simulink model "AFC_FFNN_trainlm_45_45_45_ctr_Nor_July_15"  (R2021a)
settings: Solver=VariableStepAuto  StartTime=0.0  StopTime=10.0  RelTol=1e-3
libraries: neural x140
(part 1 of 6)
settings Model: Creator=deyun  LastModifiedBy=deyun

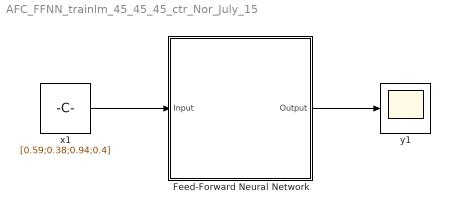
== system AFC_FFNN_trainlm_45_45_45_ctr_Nor_July_15 ==
  Feed-Forward Neural Network : Subsystem
      mask help: Feed-Forward Neural Network
      mask Display: e = 0.06;c1 = [120 150 230]/255;c2 = ([120 150 230]+0)/383;c3 = ([120 150 230]+128)/383;patch([0 1 1 0],[0 0 1 1],c1);patch([0 1 1 1-e 1-e 0+e],[0 0 1 1-e 0+e 0+e],c2);patch([0 0 1 1-e 0+e 0+e],[0 1 1 1-e 1-e 0+e],c3);plot([0 1 1 0 0],[0 0 1 1 0]);fprintf('NNET');port_label('input',1,' Input');port_label('output',1,'Output ');
  x1 : Constant  Value=[0.59;0.38;0.94;0.4]  SampleTime=1
      mask Display: e = 0.06;c1 = [120 230 180]/255;c2 = ([120 230 180]+0)/(256+128);c3 = ([120 230 180]+128)/(256+128);patch([0 1 1 0],[0 0 1 1],c1);patch([0 1 1 1-e 1-e 0+e],[0 0 1 1-e 0+e 0+e],c2);patch([0 0 1 1-e 0+e 0+e],[0 1 1 1-e 1-e 0+e],c3);plot([0 1 1 0 0],[0 0 1 1 0]);disp('Constant');
  y1 : Scope
      mask Display: e = 0.06;c1 = [120 230 180]/255;c2 = ([120 230 180]+0)/(256+128);c3 = ([120 230 180]+128)/(256+128);patch([0 1 1 0],[0 0 1 1],c1);patch([0 1 1 1-e 1-e 0+e],[0 0 1 1-e 0+e 0+e],c2);patch([0 0 1 1-e 0+e 0+e],[0 1 1 1-e 1-e 0+e],c3);plot([0 1 1 0 0],[0 0 1 1 0]);plot([0.15 0.85 0.85 0.15 0.15],[0.5 0.5 0.85 0.85 0.5]);
  wires:
  x1/1 -> Feed-Forward Neural Network/1(Input)
  Feed-Forward Neural Network/1(Output) -> y1/1

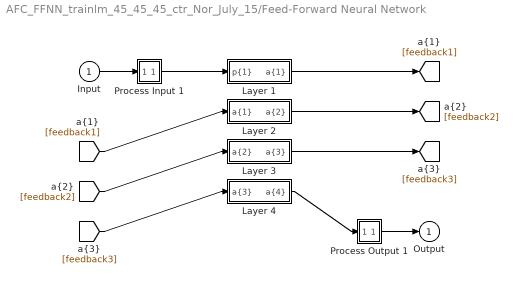
== system AFC_FFNN_trainlm_45_45_45_ctr_Nor_July_15/Feed-Forward Neural Network ==
  Input : Inport  PortDimensions=4
      mask Display: e = 0.06;c1 = [120 230 180]/255;c2 = ([120 230 180]+0)/(256+128);c3 = ([120 230 180]+128)/(256+128);patch([0 1 1 0],[0 0 1 1],c1);patch([0 1 1 1-e 1-e 0+e],[0 0 1 1-e 0+e 0+e],c2);patch([0 0 1 1-e 0+e 0+e],[0 1 1 1-e 1-e 0+e],c3);plot([0 1 1 0 0],[0 0 1 1 0]);
  Layer 1 : Subsystem
      mask Display: e = 0.06;c1 = [120 150 230]/255;c2 = ([120 150 230]+0)/383;c3 = ([120 150 230]+128)/383;patch([0 1 1 0],[0 0 1 1],c1);patch([0 1 1 1-e 1-e 0+e],[0 0 1 1-e 0+e 0+e],c2);patch([0 0 1 1-e 0+e 0+e],[0 1 1 1-e 1-e 0+e],c3);plot([0 1 1 0 0],[0 0 1 1 0]);
  Layer 2 : Subsystem
      mask Display: e = 0.06;c1 = [120 150 230]/255;c2 = ([120 150 230]+0)/383;c3 = ([120 150 230]+128)/383;patch([0 1 1 0],[0 0 1 1],c1);patch([0 1 1 1-e 1-e 0+e],[0 0 1 1-e 0+e 0+e],c2);patch([0 0 1 1-e 0+e 0+e],[0 1 1 1-e 1-e 0+e],c3);plot([0 1 1 0 0],[0 0 1 1 0]);
  Layer 3 : Subsystem
      mask Display: e = 0.06;c1 = [120 150 230]/255;c2 = ([120 150 230]+0)/383;c3 = ([120 150 230]+128)/383;patch([0 1 1 0],[0 0 1 1],c1);patch([0 1 1 1-e 1-e 0+e],[0 0 1 1-e 0+e 0+e],c2);patch([0 0 1 1-e 0+e 0+e],[0 1 1 1-e 1-e 0+e],c3);plot([0 1 1 0 0],[0 0 1 1 0]);
  Layer 4 : Subsystem
      mask Display: e = 0.06;c1 = [120 150 230]/255;c2 = ([120 150 230]+0)/383;c3 = ([120 150 230]+128)/383;patch([0 1 1 0],[0 0 1 1],c1);patch([0 1 1 1-e 1-e 0+e],[0 0 1 1-e 0+e 0+e],c2);patch([0 0 1 1-e 0+e 0+e],[0 1 1 1-e 1-e 0+e],c3);plot([0 1 1 0 0],[0 0 1 1 0]);
  Process Input 1 : Subsystem
      mask Display: e = 0.06;c1 = [120 150 230]/255;c2 = ([120 150 230]+0)/383;c3 = ([120 150 230]+128)/383;patch([0 1 1 0],[0 0 1 1],c1);patch([0 1 1 1-e 1-e 0+e],[0 0 1 1-e 0+e 0+e],c2);patch([0 0 1 1-e 0+e 0+e],[0 1 1 1-e 1-e 0+e],c3);plot([0 1 1 0 0],[0 0 1 1 0]);
  Process Output 1 : Subsystem
      mask Display: e = 0.06;c1 = [120 150 230]/255;c2 = ([120 150 230]+0)/383;c3 = ([120 150 230]+128)/383;patch([0 1 1 0],[0 0 1 1],c1);patch([0 1 1 1-e 1-e 0+e],[0 0 1 1-e 0+e 0+e],c2);patch([0 0 1 1-e 0+e 0+e],[0 1 1 1-e 1-e 0+e],c3);plot([0 1 1 0 0],[0 0 1 1 0]);
  Output : Outport  InitialOutput=0
      mask Display: e = 0.06;c1 = [120 230 180]/255;c2 = ([120 230 180]+0)/(256+128);c3 = ([120 230 180]+128)/(256+128);patch([0 1 1 0],[0 0 1 1],c1);patch([0 1 1 1-e 1-e 0+e],[0 0 1 1-e 0+e 0+e],c2);patch([0 0 1 1-e 0+e 0+e],[0 1 1 1-e 1-e 0+e],c3);plot([0 1 1 0 0],[0 0 1 1 0]);
  wires:
  Input/1 -> Process Input 1/1(x)
  Process Output 1/1(y) -> Output/1
  Process Input 1/1(p) -> Layer 1/1("p{1}")
  Layer 1/1("a{1}") -> [feedback1]
  [feedback1] -> Layer 2/1("a{1} ")
  Layer 2/1("a{2}") -> [feedback2]
  [feedback2] -> Layer 3/1("a{2} ")
  Layer 3/1("a{3}") -> [feedback3]
  [feedback3] -> Layer 4/1("a{3} ")
  Layer 4/1("a{4}") -> Process Output 1/1(a)

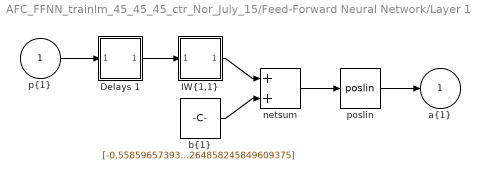
== system AFC_FFNN_trainlm_45_45_45_ctr_Nor_July_15/Feed-Forward Neural Network/Layer 1 ==
  "p{1}" : Inport  PortDimensions=4
      mask Display: e = 0.06;c1 = [120 230 180]/255;c2 = ([120 230 180]+0)/(256+128);c3 = ([120 230 180]+128)/(256+128);patch([0 1 1 0],[0 0 1 1],c1);patch([0 1 1 1-e 1-e 0+e],[0 0 1 1-e 0+e 0+e],c2);patch([0 0 1 1-e 0+e 0+e],[0 1 1 1-e 1-e 0+e],c3);plot([0 1 1 0 0],[0 0 1 1 0]);
  Delays 1 : Subsystem
      mask Display: e = 0.06;c1 = [120 150 230]/255;c2 = ([120 150 230]+0)/383;c3 = ([120 150 230]+128)/383;patch([0 1 1 0],[0 0 1 1],c1);patch([0 1 1 1-e 1-e 0+e],[0 0 1 1-e 0+e 0+e],c2);patch([0 0 1 1-e 0+e 0+e],[0 1 1 1-e 1-e 0+e],c3);plot([0 1 1 0 0],[0 0 1 1 0]);disp('0');
  "IW{1,1}" : Subsystem
      mask Display: e = 0.06;c1 = [120 150 230]/255;c2 = ([120 150 230]+0)/383;c3 = ([120 150 230]+128)/383;patch([0 1 1 0],[0 0 1 1],c1);patch([0 1 1 1-e 1-e 0+e],[0 0 1 1-e 0+e 0+e],c2);patch([0 0 1 1-e 0+e 0+e],[0 1 1 1-e 1-e 0+e],c3);plot([0 1 1 0 0],[0 0 1 1 0]);disp('W');
  "b{1}" : Constant  Value=[-0.5585965739320057910077821361483074724674224853515625;-0.77112950387139012065063070622272789478302001953125;0.22894666757716020111246280066552571952342987060546875;-0.305047379583083699827739110332913696765899658203125;-0.69451441467543661989481051932671107351779937744140625;0.39214635280524723359718564097420312464237213134765625;-0.1555721937487436756786252090023481287062168121337890625;0.274827394729951490770503141902736388146877288818359375;0.277365245819692296525005303919897414743900299072265625;-0.1524186026109950187201746985010686330497264862060546875;-0.0018307247949869154268753845826722681522369384765625;0.58822997451524916545650967236724682152271270751953125;0.55084837701463318371253308214363642036914825439453125;0.314130170445041712046219117837608791887760162353515625;-0.07693509824360840465562461076842737384140491485595703125;-0.851136421274869547914931899867951869964599609375;0.362298342175110754670441792768542654812335968017578125;0.21255578744349323816464902847656048834323883056640625;-0.3824877228684744334685774447279982268810272216796875;-0.6749591132024963524571603556978516280651092529296875;-0.63890547966722144312967657242552377283573150634765625;-0.149732930796697971675968119598110206425189971923828125;-0.933207190422134402751908055506646633148193359375;0.10402318613955320592001640989110455848276615142822265625;0.829936502547987675626472992007620632648468017578125;-0.737888972575629242811601216089911758899688720703125;0.21732415928306558772220569153432734310626983642578125;-0.1580532967861125737130123525275848805904388427734375;-1.288298758066100280217369800084270536899566650390625;-0.9481540190806569956549765265663154423236846923828125;0.942806016112406108931054404820315539836883544921875;-0.439159443551665196192601570146507583558559417724609375;0.276425093592411907916783775363001041114330291748046875;0.485464567417084047473707641984219662845134735107421875;0.295746825087029263645632681800634600222110748291015625;-0.8382271786519968070905406420934014022350311279296875;-0.1591390063283328881738043492077849805355072021484375;-0.7823304156725818803153060798649676144123077392578125;0.2224216466664273028630560702367802150547504425048828125;0.75721224172485557257772370576276443898677825927734375;-0.26127862544034818892413341018254868686199188232421875;0.1681522472301393289484394699684344232082366943359375;0.00998894613673773079653983586467802524566650390625;-0.6614665456480552929718896848498843610286712646484375;-0.838290046288482582070855642086826264858245849609375]
      mask Display: e = 0.06;c1 = [120 150 230]/255;c2 = ([120 150 230]+0)/383;c3 = ([120 150 230]+128)/383;patch([0 1 1 0],[0 0 1 1],c1);patch([0 1 1 1-e 1-e 0+e],[0 0 1 1-e 0+e 0+e],c2);patch([0 0 1 1-e 0+e 0+e],[0 1 1 1-e 1-e 0+e],c3);plot([0 1 1 0 0],[0 0 1 1 0]);disp('b');
  netsum : Sum  Inputs=2  InputSameDT=on  SaturateOnIntegerOverflow=on  OutDataTypeStr=Inherit: Same as first input
      mask Display: e = 0.06;c1 = [120 150 230]/255;c2 = ([120 150 230]+0)/383;c3 = ([120 150 230]+128)/383;patch([0 1 1 0],[0 0 1 1],c1);patch([0 1 1 1-e 1-e 0+e],[0 0 1 1-e 0+e 0+e],c2);patch([0 0 1 1-e 0+e 0+e],[0 1 1 1-e 1-e 0+e],c3);plot([0 1 1 0 0],[0 0 1 1 0]);disp('+');
  poslin : neural/Transfer Functions/poslin
      settings: SourceProductBaseCode=NN
  "a{1}" : Outport  InitialOutput=[0;0;0;0;0;0;0;0;0;0;0;0;0;0;0;0;0;0;0;0;0;0;0;0;0;0;0;0;0;0;0;0;0;0;0;0;0;0;0;0;0;0;0;0;0]
      mask Display: e = 0.06;c1 = [120 230 180]/255;c2 = ([120 230 180]+0)/(256+128);c3 = ([120 230 180]+128)/(256+128);patch([0 1 1 0],[0 0 1 1],c1);patch([0 1 1 1-e 1-e 0+e],[0 0 1 1-e 0+e 0+e],c2);patch([0 0 1 1-e 0+e 0+e],[0 1 1 1-e 1-e 0+e],c3);plot([0 1 1 0 0],[0 0 1 1 0]);
  wires:
  "p{1}"/1 -> Delays 1/1("p{1}")
  Delays 1/1("pd{1,1}") -> "IW{1,1}"/1("pd{1,1}")
  "IW{1,1}"/1("iz{1,1}") -> netsum/1
  "b{1}"/1 -> netsum/2
  netsum/1 -> poslin/1
  poslin/1 -> "a{1}"/1

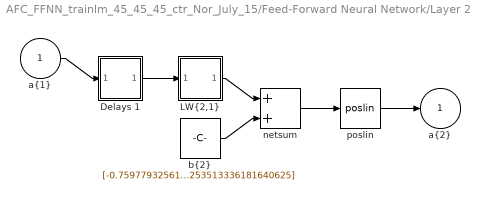
== system AFC_FFNN_trainlm_45_45_45_ctr_Nor_July_15/Feed-Forward Neural Network/Layer 2 ==
  "a{1} " : Inport  PortDimensions=45
      mask Display: e = 0.06;c1 = [120 230 180]/255;c2 = ([120 230 180]+0)/(256+128);c3 = ([120 230 180]+128)/(256+128);patch([0 1 1 0],[0 0 1 1],c1);patch([0 1 1 1-e 1-e 0+e],[0 0 1 1-e 0+e 0+e],c2);patch([0 0 1 1-e 0+e 0+e],[0 1 1 1-e 1-e 0+e],c3);plot([0 1 1 0 0],[0 0 1 1 0]);
  Delays 1 : Subsystem
      mask Display: e = 0.06;c1 = [120 150 230]/255;c2 = ([120 150 230]+0)/383;c3 = ([120 150 230]+128)/383;patch([0 1 1 0],[0 0 1 1],c1);patch([0 1 1 1-e 1-e 0+e],[0 0 1 1-e 0+e 0+e],c2);patch([0 0 1 1-e 0+e 0+e],[0 1 1 1-e 1-e 0+e],c3);plot([0 1 1 0 0],[0 0 1 1 0]);disp('0');
  "LW{2,1}" : Subsystem
      mask Display: e = 0.06;c1 = [120 150 230]/255;c2 = ([120 150 230]+0)/383;c3 = ([120 150 230]+128)/383;patch([0 1 1 0],[0 0 1 1],c1);patch([0 1 1 1-e 1-e 0+e],[0 0 1 1-e 0+e 0+e],c2);patch([0 0 1 1-e 0+e 0+e],[0 1 1 1-e 1-e 0+e],c3);plot([0 1 1 0 0],[0 0 1 1 0]);disp('W');
  "b{2}" : Constant  Value=[-0.759779325613544553874589837505482137203216552734375;0.6965202526642186864336281360010616481304168701171875;-0.861179161880855748023577689309604465961456298828125;0.279069361418990080636604034225456416606903076171875;0.7788995695670519747721982639632187783718109130859375;0.72059847295826762181292224340722896158695220947265625;0.56823299771985691375419946780311875045299530029296875;-0.814016852489903186551600811071693897247314453125;-0.25020043213131148984729179574060253798961639404296875;0.3676809986895264170669861414353363215923309326171875;-0.5664709440966280151741329973447136580944061279296875;0.02629409189089770837455262153525836765766143798828125;-0.54936854809591240123012312324135564267635345458984375;-0.133862432529689490134927609688020311295986175537109375;-0.81332808228198449906898304107016883790493011474609375;-0.75199519420301730310285392988589592278003692626953125;-1.0530530335707963818236976294429041445255279541015625;-0.3949760005903317772180116662639193236827850341796875;0.08349711700445057449559982387654599733650684356689453125;-0.5150947870913196169340153574012219905853271484375;0.80569296901346032502289062904310412704944610595703125;-0.335455649950676171311414464071276597678661346435546875;0.2177777173381762187975851929877535440027713775634765625;-0.24227916035240870673561630610493011772632598876953125;-0.7581191909009616924919328084797598421573638916015625;-0.316127694986459373271969752750010229647159576416015625;-0.7572608648365470873642379956436343491077423095703125;-0.1771784549431406896591312261080020107328891754150390625;0.6700945036965897383396395525778643786907196044921875;-0.37793060271353240420211250238935463130474090576171875;0.49989124604212953340010017200256697833538055419921875;-0.8804292366841608430405585750122554600238800048828125;-0.68894262263308225779923077425337396562099456787109375;-0.7835754927496629829164476177538745105266571044921875;-0.331990649298899709318533268742612563073635101318359375;-0.365329678636181875983623967840685509145259857177734375;-0.1674592513076313959885510485037229955196380615234375;-0.65902586680079677794452663874835707247257232666015625;-0.045949912742535292675682967455941252410411834716796875;-0.56660135380107534697202709139673970639705657958984375;0.85478289689744979540364511194638907909393310546875;0.8907503577019373341983055070159025490283966064453125;-0.7442862631882911639280564486398361623287200927734375;0.8790617462862424513758696775767020881175994873046875;-0.487941954201235095212041414924897253513336181640625]
      mask Display: e = 0.06;c1 = [120 150 230]/255;c2 = ([120 150 230]+0)/383;c3 = ([120 150 230]+128)/383;patch([0 1 1 0],[0 0 1 1],c1);patch([0 1 1 1-e 1-e 0+e],[0 0 1 1-e 0+e 0+e],c2);patch([0 0 1 1-e 0+e 0+e],[0 1 1 1-e 1-e 0+e],c3);plot([0 1 1 0 0],[0 0 1 1 0]);disp('b');
  netsum : Sum  Inputs=2  InputSameDT=on  SaturateOnIntegerOverflow=on  OutDataTypeStr=Inherit: Same as first input
      mask Display: e = 0.06;c1 = [120 150 230]/255;c2 = ([120 150 230]+0)/383;c3 = ([120 150 230]+128)/383;patch([0 1 1 0],[0 0 1 1],c1);patch([0 1 1 1-e 1-e 0+e],[0 0 1 1-e 0+e 0+e],c2);patch([0 0 1 1-e 0+e 0+e],[0 1 1 1-e 1-e 0+e],c3);plot([0 1 1 0 0],[0 0 1 1 0]);disp('+');
  poslin : neural/Transfer Functions/poslin
      settings: SourceProductBaseCode=NN
  "a{2}" : Outport  InitialOutput=[0;0;0;0;0;0;0;0;0;0;0;0;0;0;0;0;0;0;0;0;0;0;0;0;0;0;0;0;0;0;0;0;0;0;0;0;0;0;0;0;0;0;0;0;0]
      mask Display: e = 0.06;c1 = [120 230 180]/255;c2 = ([120 230 180]+0)/(256+128);c3 = ([120 230 180]+128)/(256+128);patch([0 1 1 0],[0 0 1 1],c1);patch([0 1 1 1-e 1-e 0+e],[0 0 1 1-e 0+e 0+e],c2);patch([0 0 1 1-e 0+e 0+e],[0 1 1 1-e 1-e 0+e],c3);plot([0 1 1 0 0],[0 0 1 1 0]);
  wires:
  "a{1} "/1 -> Delays 1/1("p{2}")
  Delays 1/1("pd{2,1}") -> "LW{2,1}"/1("ad{2,1}")
  "LW{2,1}"/1("lz{2,1}") -> netsum/1
  "b{2}"/1 -> netsum/2
  netsum/1 -> poslin/1
  poslin/1 -> "a{2}"/1

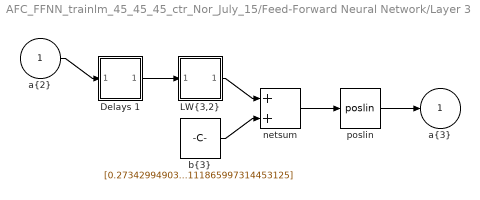
== system AFC_FFNN_trainlm_45_45_45_ctr_Nor_July_15/Feed-Forward Neural Network/Layer 3 ==
  "a{2} " : Inport  PortDimensions=45
      mask Display: e = 0.06;c1 = [120 230 180]/255;c2 = ([120 230 180]+0)/(256+128);c3 = ([120 230 180]+128)/(256+128);patch([0 1 1 0],[0 0 1 1],c1);patch([0 1 1 1-e 1-e 0+e],[0 0 1 1-e 0+e 0+e],c2);patch([0 0 1 1-e 0+e 0+e],[0 1 1 1-e 1-e 0+e],c3);plot([0 1 1 0 0],[0 0 1 1 0]);
  Delays 1 : Subsystem
      mask Display: e = 0.06;c1 = [120 150 230]/255;c2 = ([120 150 230]+0)/383;c3 = ([120 150 230]+128)/383;patch([0 1 1 0],[0 0 1 1],c1);patch([0 1 1 1-e 1-e 0+e],[0 0 1 1-e 0+e 0+e],c2);patch([0 0 1 1-e 0+e 0+e],[0 1 1 1-e 1-e 0+e],c3);plot([0 1 1 0 0],[0 0 1 1 0]);disp('0');
  "LW{3,2}" : Subsystem
      mask Display: e = 0.06;c1 = [120 150 230]/255;c2 = ([120 150 230]+0)/383;c3 = ([120 150 230]+128)/383;patch([0 1 1 0],[0 0 1 1],c1);patch([0 1 1 1-e 1-e 0+e],[0 0 1 1-e 0+e 0+e],c2);patch([0 0 1 1-e 0+e 0+e],[0 1 1 1-e 1-e 0+e],c3);plot([0 1 1 0 0],[0 0 1 1 0]);disp('W');
  "b{3}" : Constant  Value=[0.2734299490328331305732945111230947077274322509765625;0.253212645186324747381689803660265170037746429443359375;0.93467329178748126405906759828212670981884002685546875;0.85424049495533072029473942166077904403209686279296875;0.370732482252811246237200748510076664388179779052734375;0.58575586111893096497027499935938976705074310302734375;-0.57222729704926555971411517020897008478641510009765625;0.402075725104235726092838376644067466259002685546875;0.77510392535672212321884444463648833334445953369140625;0.89750677439359172193888980473275296390056610107421875;-0.53893848136911326474063343994203023612499237060546875;-0.447084590177655893938890585559420287609100341796875;-0.16971363346798085114386367422412149608135223388671875;-0.1253386080403514346581772542776889167726039886474609375;0.7324385856904609415352069845539517700672149658203125;-0.1718566614749994225785911794446292333304882049560546875;-0.649121257858855216227311757393181324005126953125;0.0020706443178506819292883367467084099189378321170806884765625;0.14280132148982105366741279794950969517230987548828125;-0.400326950100625911233009901479817926883697509765625;-0.09611968684726655831607189384158118627965450286865234375;-0.86780297012492602082289749887422658503055572509765625;-0.22662709591045449020185742483590729534626007080078125;-0.049925910120531102887042607108014635741710662841796875;0.957436543865733735714229624136351048946380615234375;0.557449966972769939133058869629167020320892333984375;-0.28645987977858933248853645636700093746185302734375;0.1261192693375135787103857865076861344277858734130859375;-0.5205296579813223356580920153646729886531829833984375;0.30033442526422593488177881226874887943267822265625;-0.17988670535213813206354416251997463405132293701171875;0.88536176329107918459015991174965165555477142333984375;0.52550652298814781726576939036021940410137176513671875;0.55963934687581906590736480211489833891391754150390625;0.1453135731776866723663488301099278032779693603515625;0.5122265681069091414201466250233352184295654296875;-0.3700450504693375552989209609222598373889923095703125;0.0395997938226071710676734483058680780231952667236328125;0.741921262418416826989187029539607465267181396484375;-0.1478710785470286614984303241726593114435672760009765625;0.3344458719405338786856418664683587849140167236328125;-0.562784675088596753056435773032717406749725341796875;0.6146888018342695492179927896359004080295562744140625;0.41510836491622049582161935177282430231571197509765625;0.885843136212703274878776937839575111865997314453125]
      mask Display: e = 0.06;c1 = [120 150 230]/255;c2 = ([120 150 230]+0)/383;c3 = ([120 150 230]+128)/383;patch([0 1 1 0],[0 0 1 1],c1);patch([0 1 1 1-e 1-e 0+e],[0 0 1 1-e 0+e 0+e],c2);patch([0 0 1 1-e 0+e 0+e],[0 1 1 1-e 1-e 0+e],c3);plot([0 1 1 0 0],[0 0 1 1 0]);disp('b');
  netsum : Sum  Inputs=2  InputSameDT=on  SaturateOnIntegerOverflow=on  OutDataTypeStr=Inherit: Same as first input
      mask Display: e = 0.06;c1 = [120 150 230]/255;c2 = ([120 150 230]+0)/383;c3 = ([120 150 230]+128)/383;patch([0 1 1 0],[0 0 1 1],c1);patch([0 1 1 1-e 1-e 0+e],[0 0 1 1-e 0+e 0+e],c2);patch([0 0 1 1-e 0+e 0+e],[0 1 1 1-e 1-e 0+e],c3);plot([0 1 1 0 0],[0 0 1 1 0]);disp('+');
  poslin : neural/Transfer Functions/poslin
      settings: SourceProductBaseCode=NN
  "a{3}" : Outport  InitialOutput=[0;0;0;0;0;0;0;0;0;0;0;0;0;0;0;0;0;0;0;0;0;0;0;0;0;0;0;0;0;0;0;0;0;0;0;0;0;0;0;0;0;0;0;0;0]
      mask Display: e = 0.06;c1 = [120 230 180]/255;c2 = ([120 230 180]+0)/(256+128);c3 = ([120 230 180]+128)/(256+128);patch([0 1 1 0],[0 0 1 1],c1);patch([0 1 1 1-e 1-e 0+e],[0 0 1 1-e 0+e 0+e],c2);patch([0 0 1 1-e 0+e 0+e],[0 1 1 1-e 1-e 0+e],c3);plot([0 1 1 0 0],[0 0 1 1 0]);
  wires:
  "a{2} "/1 -> Delays 1/1("p{3}")
  Delays 1/1("pd{3,2}") -> "LW{3,2}"/1("ad{3,2}")
  "LW{3,2}"/1("lz{3,2}") -> netsum/1
  "b{3}"/1 -> netsum/2
  netsum/1 -> poslin/1
  poslin/1 -> "a{3}"/1

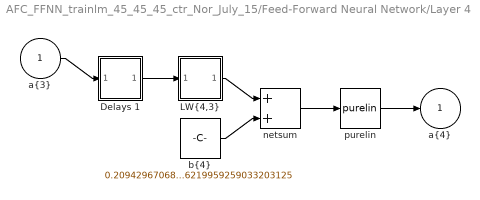
== system AFC_FFNN_trainlm_45_45_45_ctr_Nor_July_15/Feed-Forward Neural Network/Layer 4 ==
  "a{3} " : Inport  PortDimensions=45
      mask Display: e = 0.06;c1 = [120 230 180]/255;c2 = ([120 230 180]+0)/(256+128);c3 = ([120 230 180]+128)/(256+128);patch([0 1 1 0],[0 0 1 1],c1);patch([0 1 1 1-e 1-e 0+e],[0 0 1 1-e 0+e 0+e],c2);patch([0 0 1 1-e 0+e 0+e],[0 1 1 1-e 1-e 0+e],c3);plot([0 1 1 0 0],[0 0 1 1 0]);
  Delays 1 : Subsystem
      mask Display: e = 0.06;c1 = [120 150 230]/255;c2 = ([120 150 230]+0)/383;c3 = ([120 150 230]+128)/383;patch([0 1 1 0],[0 0 1 1],c1);patch([0 1 1 1-e 1-e 0+e],[0 0 1 1-e 0+e 0+e],c2);patch([0 0 1 1-e 0+e 0+e],[0 1 1 1-e 1-e 0+e],c3);plot([0 1 1 0 0],[0 0 1 1 0]);disp('0');
  "LW{4,3}" : Subsystem
      mask Display: e = 0.06;c1 = [120 150 230]/255;c2 = ([120 150 230]+0)/383;c3 = ([120 150 230]+128)/383;patch([0 1 1 0],[0 0 1 1],c1);patch([0 1 1 1-e 1-e 0+e],[0 0 1 1-e 0+e 0+e],c2);patch([0 0 1 1-e 0+e 0+e],[0 1 1 1-e 1-e 0+e],c3);plot([0 1 1 0 0],[0 0 1 1 0]);disp('W');
  "b{4}" : Constant  Value=0.2094296706820160391959717571808141656219959259033203125
      mask Display: e = 0.06;c1 = [120 150 230]/255;c2 = ([120 150 230]+0)/383;c3 = ([120 150 230]+128)/383;patch([0 1 1 0],[0 0 1 1],c1);patch([0 1 1 1-e 1-e 0+e],[0 0 1 1-e 0+e 0+e],c2);patch([0 0 1 1-e 0+e 0+e],[0 1 1 1-e 1-e 0+e],c3);plot([0 1 1 0 0],[0 0 1 1 0]);disp('b');
  netsum : Sum  Inputs=2  InputSameDT=on  SaturateOnIntegerOverflow=on  OutDataTypeStr=Inherit: Same as first input
      mask Display: e = 0.06;c1 = [120 150 230]/255;c2 = ([120 150 230]+0)/383;c3 = ([120 150 230]+128)/383;patch([0 1 1 0],[0 0 1 1],c1);patch([0 1 1 1-e 1-e 0+e],[0 0 1 1-e 0+e 0+e],c2);patch([0 0 1 1-e 0+e 0+e],[0 1 1 1-e 1-e 0+e],c3);plot([0 1 1 0 0],[0 0 1 1 0]);disp('+');
  purelin : neural/Transfer Functions/purelin
  "a{4}" : Outport  InitialOutput=0
      mask Display: e = 0.06;c1 = [120 230 180]/255;c2 = ([120 230 180]+0)/(256+128);c3 = ([120 230 180]+128)/(256+128);patch([0 1 1 0],[0 0 1 1],c1);patch([0 1 1 1-e 1-e 0+e],[0 0 1 1-e 0+e 0+e],c2);patch([0 0 1 1-e 0+e 0+e],[0 1 1 1-e 1-e 0+e],c3);plot([0 1 1 0 0],[0 0 1 1 0]);
  wires:
  "a{3} "/1 -> Delays 1/1("p{4}")
  Delays 1/1("pd{4,3}") -> "LW{4,3}"/1("ad{4,3}")
  "LW{4,3}"/1("lz{4,3}") -> netsum/1
  "b{4}"/1 -> netsum/2
  netsum/1 -> purelin/1
  purelin/1 -> "a{4}"/1

== system AFC_FFNN_trainlm_45_45_45_ctr_Nor_July_15/Feed-Forward Neural Network/Process Input 1 ==
  x : Inport  PortDimensions=4
      mask Display: e = 0.06;c1 = [120 230 180]/255;c2 = ([120 230 180]+0)/(256+128);c3 = ([120 230 180]+128)/(256+128);patch([0 1 1 0],[0 0 1 1],c1);patch([0 1 1 1-e 1-e 0+e],[0 0 1 1-e 0+e 0+e],c2);patch([0 0 1 1-e 0+e 0+e],[0 1 1 1-e 1-e 0+e],c3);plot([0 1 1 0 0],[0 0 1 1 0]);
  p : Outport  PortDimensions=4
      mask Display: e = 0.06;c1 = [120 230 180]/255;c2 = ([120 230 180]+0)/(256+128);c3 = ([120 230 180]+128)/(256+128);patch([0 1 1 0],[0 0 1 1],c1);patch([0 1 1 1-e 1-e 0+e],[0 0 1 1-e 0+e 0+e],c2);patch([0 0 1 1-e 0+e 0+e],[0 1 1 1-e 1-e 0+e],c3);plot([0 1 1 0 0],[0 0 1 1 0]);
  wires:
  x/1 -> p/1

== system AFC_FFNN_trainlm_45_45_45_ctr_Nor_July_15/Feed-Forward Neural Network/Process Output 1 ==
  a : Inport  PortDimensions=1
      mask Display: e = 0.06;c1 = [120 230 180]/255;c2 = ([120 230 180]+0)/(256+128);c3 = ([120 230 180]+128)/(256+128);patch([0 1 1 0],[0 0 1 1],c1);patch([0 1 1 1-e 1-e 0+e],[0 0 1 1-e 0+e 0+e],c2);patch([0 0 1 1-e 0+e 0+e],[0 1 1 1-e 1-e 0+e],c3);plot([0 1 1 0 0],[0 0 1 1 0]);
  y : Outport  PortDimensions=1
      mask Display: e = 0.06;c1 = [120 230 180]/255;c2 = ([120 230 180]+0)/(256+128);c3 = ([120 230 180]+128)/(256+128);patch([0 1 1 0],[0 0 1 1],c1);patch([0 1 1 1-e 1-e 0+e],[0 0 1 1-e 0+e 0+e],c2);patch([0 0 1 1-e 0+e 0+e],[0 1 1 1-e 1-e 0+e],c3);plot([0 1 1 0 0],[0 0 1 1 0]);
  wires:
  a/1 -> y/1

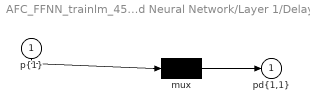
== system AFC_FFNN_trainlm_45_45_45_ctr_Nor_July_15/Feed-Forward Neural Network/Layer 1/Delays 1 ==
  "p{1}" : Inport  PortDimensions=4
      mask Display: e = 0.06;c1 = [120 230 180]/255;c2 = ([120 230 180]+0)/(256+128);c3 = ([120 230 180]+128)/(256+128);patch([0 1 1 0],[0 0 1 1],c1);patch([0 1 1 1-e 1-e 0+e],[0 0 1 1-e 0+e 0+e],c2);patch([0 0 1 1-e 0+e 0+e],[0 1 1 1-e 1-e 0+e],c3);plot([0 1 1 0 0],[0 0 1 1 0]);
  mux : Mux  Inputs=1
      mask Display: e = 0.06;c1 = [120 150 230]/255;c2 = ([120 150 230]+0)/383;c3 = ([120 150 230]+128)/383;patch([0 1 1 0],[0 0 1 1],c1);patch([0 1 1 1-e 1-e 0+e],[0 0 1 1-e 0+e 0+e],c2);patch([0 0 1 1-e 0+e 0+e],[0 1 1 1-e 1-e 0+e],c3);plot([0 1 1 0 0],[0 0 1 1 0]);disp('Mux')
  "pd{1,1}" : Outport
      mask Display: e = 0.06;c1 = [120 230 180]/255;c2 = ([120 230 180]+0)/(256+128);c3 = ([120 230 180]+128)/(256+128);patch([0 1 1 0],[0 0 1 1],c1);patch([0 1 1 1-e 1-e 0+e],[0 0 1 1-e 0+e 0+e],c2);patch([0 0 1 1-e 0+e 0+e],[0 1 1 1-e 1-e 0+e],c3);plot([0 1 1 0 0],[0 0 1 1 0]);
  wires:
  "p{1}"/1 -> mux/1
  mux/1 -> "pd{1,1}"/1
